simulink model "untitled"  (R2024a)
settings: Solver=FixedStepAuto  StartTime=0.0  StopTime=10  FixedStep=0.001  RelTol=1e-3
values from neighbouring files (symbols this model uses):
  cM = 2.925e-9    (= 2.925e-09)    [untitled1.m]
  CR = 80.584    [untitled1.m]
  cT = 1.4865e-7    (= 1.4865e-07)    [untitled1.m]
  d_x = 0.08257    [untitled1.m]
  d_y = 0.13505    [untitled1.m]
  g = 9.81    [untitled1.m]
  Ix = 0.0095    [untitled1.m]
  Iy = 0.0095    [untitled1.m]
  Iz = 0.019    [untitled1.m]
  K = cM/cT    (= 0.0196770938446)    [untitled1.m]
  Kvxd = 10    [untitled1.m]
  Kvxi = 0.001    [untitled1.m]
  Kvxp = 5    [untitled1.m]
  Kvyd = 10    [untitled1.m]
  Kvyi = 0.001    [untitled1.m]
  Kvyp = 5    [untitled1.m]
  Kvzd = 0.1    [untitled1.m]
  Kvzi = 0.01    [untitled1.m]
  Kvzp = 10    [untitled1.m]
  m = 2    [untitled1.m]
  Tm = 0.03    [untitled1.m]
  wb = 976.2    [untitled1.m]
undefined symbols (not defined in the file or in its folder): Kvpitchd, Kvpitchi, Kvpitchn, Kvpitchp, Kvrolld, Kvrolli, Kvrolln, Kvrollp, Kvyawd, Kvyawi, Kvyawn, Kvyawp, Kzp, magnitude
libraries: slpidlib x6
settings Model: Creator=user  LastModifiedBy=User
settings DataIOCC: ReturnWorkspaceOutputs=off

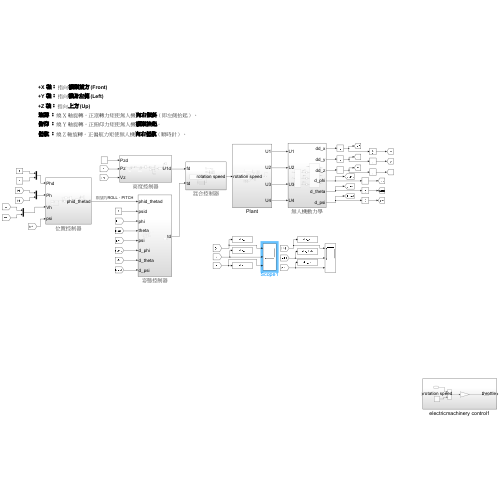
[thumbnail: Simulink's stored preview of the top-level diagram]
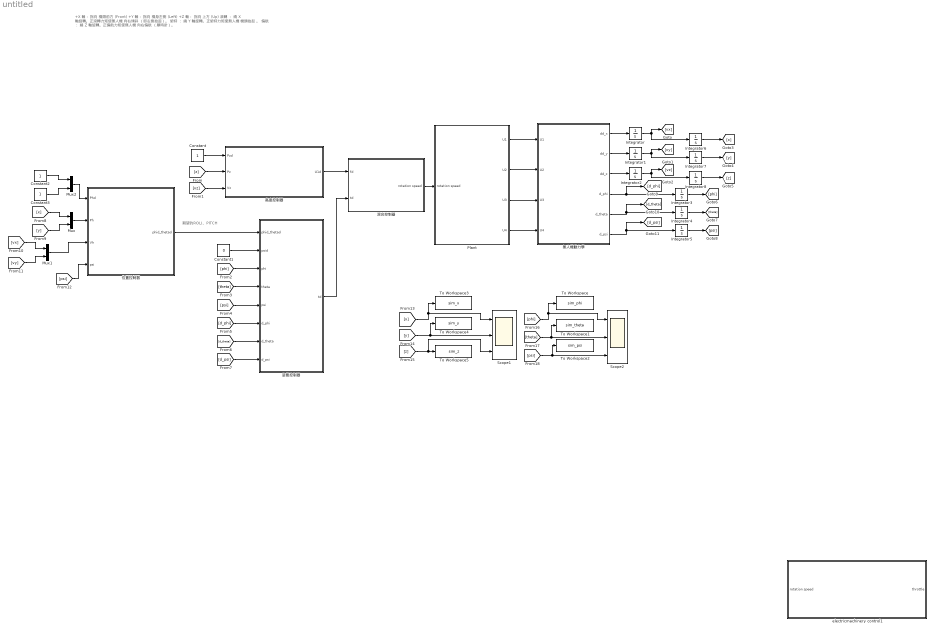
== system untitled ==
  note: +X 軸： 指向 機頭前方 (Front)
      | +Y 軸： 指向 機身左側 (Left)
      | +Z 軸： 指向 上方 (Up)
      | 滾轉 ： 繞 X 軸旋轉。正滾轉力矩使無人機 向右傾斜 （即左側抬起）。
      | 俯仰 ： 繞 Y 軸旋轉。正俯仰力矩使無人機 機頭抬起 。
      | 偏航 ： 繞 Z 軸旋轉。正偏航力矩使無人機 向右偏航 （順時針）。
  note: 期望的ROLL、PITCH
  Constant : Constant
  Constant1 : Constant  Value=0
  Constant2 : Constant
  Constant3 : Constant
  Integrator{,1..8} (9 alike) : Integrator
  Mux : Mux  Inputs=2
  Mux1 : Mux  Inputs=2
  Mux2 : Mux  Inputs=2
  Plant : Subsystem
  Scope1 : Scope  NumInputPorts=3
  Scope2 : Scope  NumInputPorts=3
  To Workspace : ToWorkspace  VariableName=sim_phi  SampleTime=-1
  To Workspace1 : ToWorkspace  VariableName=sim_theta  SampleTime=-1
  To Workspace2 : ToWorkspace  VariableName=sim_psi  SampleTime=-1
  To Workspace3 : ToWorkspace  VariableName=sim_x  SampleTime=-1
  To Workspace4 : ToWorkspace  VariableName=sim_y  SampleTime=-1
  To Workspace5 : ToWorkspace  VariableName=sim_z  SampleTime=-1
  electricmachinery control1 : Subsystem
  位置控制器 : Subsystem
  姿態控制器 : Subsystem
  混合控制器 : Subsystem
  無人機動力學 : Subsystem
  高度控制器 : Subsystem
  wires:
  無人機動力學/1(dd_x) -> Integrator/1
  無人機動力學/2(dd_y) -> Integrator1/1
  無人機動力學/3(dd_z) -> Integrator2/1
  無人機動力學/4(d_phi) -> Integrator3/1, [d_phi]
  無人機動力學/5(d_theta) -> Integrator4/1, [d_theta]
  無人機動力學/6(d_psi) -> Integrator5/1, [d_psi]
  Integrator/1 -> Integrator6/1, [vx]
  Integrator1/1 -> Integrator7/1, [vy]
  Integrator2/1 -> Integrator8/1, [vz]
  Integrator8/1 -> [z]
  Integrator7/1 -> [y]
  Integrator6/1 -> [x]
  Integrator3/1 -> [phi]
  Integrator4/1 -> [theta]
  Integrator5/1 -> [psi]
  高度控制器/1(U1d) -> 混合控制器/1(fd)
  Constant/1 -> 高度控制器/1(Pzd)
  [z] -> 高度控制器/2(Pz)
  [vz] -> 高度控制器/3(Vz)
  位置控制器/1(phid_thetad) -> 姿態控制器/1(phid_thetad)
  Constant1/1 -> 姿態控制器/2(psid)
  [phi] -> 姿態控制器/3(phi)
  [theta] -> 姿態控制器/4(theta)
  [d_psi] -> 姿態控制器/8(d_psi)
  [psi] -> 姿態控制器/5(psi)
  [d_phi] -> 姿態控制器/6(d_phi)
  [d_theta] -> 姿態控制器/7(d_theta)
  姿態控制器/1(td) -> 混合控制器/2(td)
  Mux/1 -> 位置控制器/2(Ph)
  [x] -> Mux/1
  [y] -> Mux/2
  [vx] -> Mux1/1
  [vy] -> Mux1/2
  Mux1/1 -> 位置控制器/3(Vh)
  [psi] -> 位置控制器/4(psi)
  Constant2/1 -> Mux2/1
  Constant3/1 -> Mux2/2
  Mux2/1 -> 位置控制器/1(Phd)
  [y] -> To Workspace4/1, Scope1/2
  [x] -> Scope1/1, To Workspace3/1
  [z] -> To Workspace5/1, Scope1/3
  [phi] -> To Workspace/1, Scope2/1
  [theta] -> To Workspace1/1, Scope2/2
  [psi] -> To Workspace2/1, Scope2/3
  混合控制器/1(rotation speed) -> Plant/1(rotation speed)
  Plant/4(U4) -> 無人機動力學/4(U4)
  Plant/3(U3) -> 無人機動力學/3(U3)
  Plant/2(U2) -> 無人機動力學/2(U2)
  Plant/1(U1) -> 無人機動力學/1(U1)

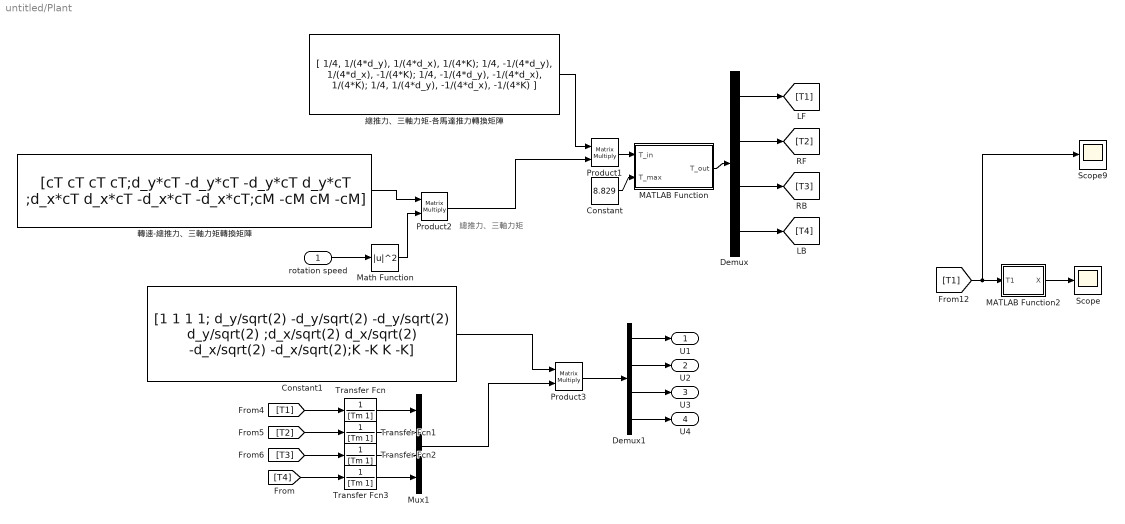
== system untitled/Plant ==
  note: 總推力、三軸力矩
  rotation speed : Inport
  Constant : Constant  Value=8.829
  Constant1 : Constant  Value=[1 1 1 1; d_y/sqrt(2) -d_y/sqrt(2) -d_y/sqrt(2) d_y/sqrt(2) ;d_x/sqrt(2) d_x/sqrt(2) -d_x/sqrt(2) -d_x/sqrt(2);K -K K -K]
  Demux : Demux
  Demux1 : Demux
  MATLAB Function : MATLAB Function  TreatAsAtomicUnit=on
  MATLAB Function2 : MATLAB Function  TreatAsAtomicUnit=on
  Math Function : Math  Operator=magnitude^2
  Mux1 : Mux
  Product1 : Product  Multiplication=Matrix(*)
  Product2 : Product  Multiplication=Matrix(*)
  Product3 : Product  Multiplication=Matrix(*)
  Scope : Scope
  Scope9 : Scope
  Transfer Fcn{,1..3} (4 alike) : TransferFcn  Denominator=[Tm 1]
  總推力、三軸力矩-各馬達推力轉換矩陣 : Constant  Value=|
      | [ 1/4,    1/(4*d_y),    1/(4*d_x),    1/(4*K);
      |   1/4,   -1/(4*d_y),    1/(4*d_x),   -1/(4*K);
      |   1/4,   -1/(4*d_y),   -1/(4*d_x),    1/(4*K);
      |   1/4,    1/(4*d_y),   -1/(4*d_x),   -1/(4*K) ]
  轉速-總推力、三軸力矩轉換矩陣 : Constant  Value=[cT cT cT cT;d_y*cT -d_y*cT -d_y*cT d_y*cT ;d_x*cT d_x*cT -d_x*cT -d_x*cT;cM -cM cM -cM]
  U1 : Outport
  U2 : Outport  Port=2
  U3 : Outport  Port=3
  U4 : Outport  Port=4
  wires:
  Constant1/1 -> Product3/1
  [T1] -> Scope9/1, MATLAB Function2/1(T1)
  MATLAB Function2/1(X) -> Scope/1
  Product3/1 -> Demux1/1
  Demux1/3 -> U3/1
  Demux1/4 -> U4/1
  Demux1/1 -> U1/1
  Demux1/2 -> U2/1
  Demux/1 -> [T1]
  Demux/2 -> [T2]
  Demux/3 -> [T3]
  Demux/4 -> [T4]
  總推力、三軸力矩-各馬達推力轉換矩陣/1 -> Product1/1
  轉速-總推力、三軸力矩轉換矩陣/1 -> Product2/1
  Transfer Fcn/1 -> Mux1/1
  Transfer Fcn1/1 -> Mux1/2
  Transfer Fcn2/1 -> Mux1/3
  Transfer Fcn3/1 -> Mux1/4
  Product2/1 -> Product1/2
  rotation speed/1 -> Math Function/1
  [T1] -> Transfer Fcn/1
  [T2] -> Transfer Fcn1/1
  [T3] -> Transfer Fcn2/1
  [T4] -> Transfer Fcn3/1
  Math Function/1 -> Product2/2
  Mux1/1 -> Product3/2
  MATLAB Function/1(T_out) -> Demux/1
  Product1/1 -> MATLAB Function/1(T_in)
  Constant/1 -> MATLAB Function/2(T_max)

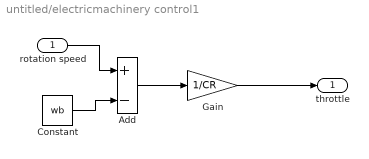
== system untitled/electricmachinery control1 ==
  rotation speed : Inport
  Add : Sum  Inputs=+-
  Constant : Constant  Value=wb
  Gain : Gain  Gain=1/CR
  throttle : Outport
  wires:
  Add/1 -> Gain/1
  rotation speed/1 -> Add/1
  Constant/1 -> Add/2
  Gain/1 -> throttle/1

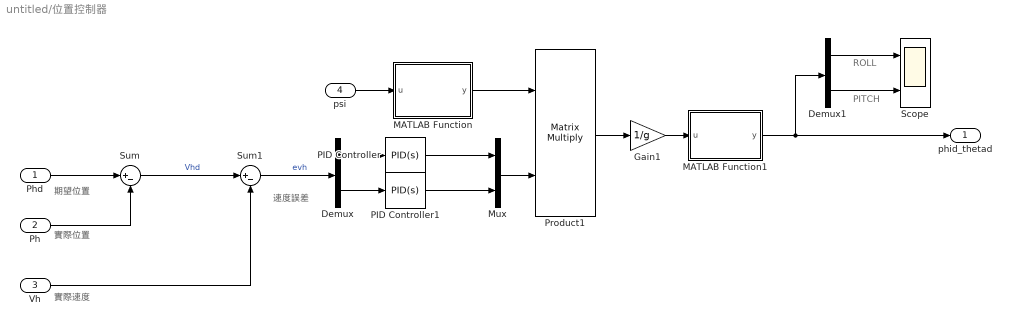
== system untitled/位置控制器 ==
  note: ROLL
  note: 期望位置
  note: 實際位置
  note: 實際速度
  note: 速度誤差
  note: PITCH
  Phd : Inport
  Ph : Inport  Port=2
  Vh : Inport  Port=3
  psi : Inport  Port=4
  Demux : Demux  Outputs=2
  Demux1 : Demux  Outputs=2
  Gain1 : Gain  Gain=1/g
  MATLAB Function : MATLAB Function  TreatAsAtomicUnit=on
  MATLAB Function1 : MATLAB Function  TreatAsAtomicUnit=on
  Mux : Mux  Inputs=2
  PID Controller : slpidlib/PID Controller  Controller=PID  Form=Parallel  TimeDomain=Continuous-time  UseExternalTs=off  SampleTime=-1  IntegratorMethod=Forward Euler  FilterMethod=Forward Euler  ControllerParametersSource=internal  P=Kvxp  I=Kvxi  UseKiTs=off  D=Kvxd  UseExternalDerivativeSource=off  N=100  UseFilter=on  TunerSelectOption=Transfer Function Based (PID Tuner App)  InitialConditionSource=internal  InitialConditionForIntegrator=0  InitialConditionForFilter=0  DifferentiatorICPrevScaledInput=0  ExternalReset=none  TrackingMode=off  Kt=1  LimitOutput=off  SatLimitsSource=internal  UpperSaturationLimit=inf  LowerSaturationLimit=-inf  LinearizeAsGain=on  AntiWindupMode=none  Kb=1  LimitIntegrator=off  UpperIntegratorSaturationLimit=inf  LowerIntegratorSaturationLimit=-inf  POutMin=[]  POutMax=[]  IOutMin=[]  IOutMax=[]  DOutMin=[]  DOutMax=[]  NOutMin=[]  NOutMax=[]  SumOutMin=[]  SumOutMax=[]  SaturationOutMin=[]  SaturationOutMax=[]  PParamMin=[]  PParamMax=[]  IParamMin=[]  IParamMax=[]  DParamMin=[]  DParamMax=[]  NParamMin=[]  NParamMax=[]  KbParamMin=[]  KbParamMax=[]  KtParamMin=[]  KtParamMax=[]  KbOutMin=[]  KbOutMax=[]  KtOutMin=[]  KtOutMax=[]  IntegratorOutMin=[]  IntegratorOutMax=[]  FilterOutMin=[]  FilterOutMax=[]  SumI1OutMin=[]  SumI1OutMax=[]  SumI2OutMin=[]  SumI2OutMax=[]  SumI3OutMin=[]  SumI3OutMax=[]  SumI4OutMin=[]  SumI4OutMax=[]  SumDOutMin=[]  SumDOutMax=[]  DifferentiatorOutMin=[]  DifferentiatorOutMax=[]  FilterDiffOutCoefMin=[]  FilterDiffOutCoefMax=[]  ReciprocalOutMin=[]  ReciprocalOutMax=[]  SumDenOutMin=[]  SumDenOutMax=[]  SumNumOutMin=[]  SumNumOutMax=[]  DivideOutMin=[]  DivideOutMax=[]  UdiffTsProdOutMin=[]  UdiffTsProdOutMax=[]  NTsProdOutMin=[]  NTsProdOutMax=[]  UintegralTsProdOutMin=[]  UintegralTsProdOutMax=[]  UngainTsProdOutMin=[]  UngainTsProdOutMax=[]  ClampingZeroOutDataTypeStr=Inherit: Inherit via back propagation  ClampingZeroOutMin=[]  ClampingZeroOutMax=[]  FilterDenConstantOutDataTypeStr=Inherit: Inherit via back propagation  FilterDenConstantOutMin=[]  FilterDenConstantOutMax=[]  PCopyOutDataTypeStr=Inherit: Inherit via back propagation  PCopyOutMin=[]  PCopyOutMax=[]  NCopyOutDataTypeStr=Inherit: Inherit via back propagation  NCopyOutMin=[]  NCopyOutMax=[]  IntegratorContinuousStateAttributes=''  IntegratorStateMustResolveToSignalObject=off  IntegratorRTWStateStorageClass=Auto  FilterContinuousStateAttributes=''  FilterStateMustResolveToSignalObject=off  FilterRTWStateStorageClass=Auto  ParallelPVariant=InternalParameters  IdealPVariant=Disabled  IVariant=InternalParameters  DVariant=InternalParameters  IntegratorVariant=Continuous  SatVariant=Disabled  AWVariant=Passthrough  PCopyVariant=Disabled  TRVariant=Disabled  FdbkBlocksVariant=Forward  IdealPFdbkVariant=Disabled  SatFdbkVariant=Disabled  DerivativeFilterVariant=ContFilter  NVariant=InternalParameters  NCopyVariant=Disabled  FilterICVariant=InternalICsFilter  IntegratorICVariant=InternalICs  ExternalResetVariant=Disabled  TRSumVariant=Passthrough  SumFdbkVariant=Disabled  SumVariant=Sum_PID  TsampFilterVariant=InternalTs  TsampNgainVariant=Passthrough  TsampIntegralVariant=Disabled_SignalSpec  ExternalSaturationOutDataTypeStr=Inherit: Same as second input  DerivativeSourceVariant=ErrorSignal
  PID Controller1 : slpidlib/PID Controller  Controller=PID  Form=Parallel  TimeDomain=Continuous-time  UseExternalTs=off  SampleTime=-1  IntegratorMethod=Forward Euler  FilterMethod=Forward Euler  ControllerParametersSource=internal  P=Kvyp  I=Kvyi  UseKiTs=off  D=Kvyd  UseExternalDerivativeSource=off  N=100  UseFilter=on  TunerSelectOption=Transfer Function Based (PID Tuner App)  InitialConditionSource=internal  InitialConditionForIntegrator=0  InitialConditionForFilter=0  DifferentiatorICPrevScaledInput=0  ExternalReset=none  TrackingMode=off  Kt=1  LimitOutput=off  SatLimitsSource=internal  UpperSaturationLimit=inf  LowerSaturationLimit=-inf  LinearizeAsGain=on  AntiWindupMode=none  Kb=1  LimitIntegrator=off  UpperIntegratorSaturationLimit=inf  LowerIntegratorSaturationLimit=-inf  POutMin=[]  POutMax=[]  IOutMin=[]  IOutMax=[]  DOutMin=[]  DOutMax=[]  NOutMin=[]  NOutMax=[]  SumOutMin=[]  SumOutMax=[]  SaturationOutMin=[]  SaturationOutMax=[]  PParamMin=[]  PParamMax=[]  IParamMin=[]  IParamMax=[]  DParamMin=[]  DParamMax=[]  NParamMin=[]  NParamMax=[]  KbParamMin=[]  KbParamMax=[]  KtParamMin=[]  KtParamMax=[]  KbOutMin=[]  KbOutMax=[]  KtOutMin=[]  KtOutMax=[]  IntegratorOutMin=[]  IntegratorOutMax=[]  FilterOutMin=[]  FilterOutMax=[]  SumI1OutMin=[]  SumI1OutMax=[]  SumI2OutMin=[]  SumI2OutMax=[]  SumI3OutMin=[]  SumI3OutMax=[]  SumI4OutMin=[]  SumI4OutMax=[]  SumDOutMin=[]  SumDOutMax=[]  DifferentiatorOutMin=[]  DifferentiatorOutMax=[]  FilterDiffOutCoefMin=[]  FilterDiffOutCoefMax=[]  ReciprocalOutMin=[]  ReciprocalOutMax=[]  SumDenOutMin=[]  SumDenOutMax=[]  SumNumOutMin=[]  SumNumOutMax=[]  DivideOutMin=[]  DivideOutMax=[]  UdiffTsProdOutMin=[]  UdiffTsProdOutMax=[]  NTsProdOutMin=[]  NTsProdOutMax=[]  UintegralTsProdOutMin=[]  UintegralTsProdOutMax=[]  UngainTsProdOutMin=[]  UngainTsProdOutMax=[]  ClampingZeroOutDataTypeStr=Inherit: Inherit via back propagation  ClampingZeroOutMin=[]  ClampingZeroOutMax=[]  FilterDenConstantOutDataTypeStr=Inherit: Inherit via back propagation  FilterDenConstantOutMin=[]  FilterDenConstantOutMax=[]  PCopyOutDataTypeStr=Inherit: Inherit via back propagation  PCopyOutMin=[]  PCopyOutMax=[]  NCopyOutDataTypeStr=Inherit: Inherit via back propagation  NCopyOutMin=[]  NCopyOutMax=[]  IntegratorContinuousStateAttributes=''  IntegratorStateMustResolveToSignalObject=off  IntegratorRTWStateStorageClass=Auto  FilterContinuousStateAttributes=''  FilterStateMustResolveToSignalObject=off  FilterRTWStateStorageClass=Auto  ParallelPVariant=InternalParameters  IdealPVariant=Disabled  IVariant=InternalParameters  DVariant=InternalParameters  IntegratorVariant=Continuous  SatVariant=Disabled  AWVariant=Passthrough  PCopyVariant=Disabled  TRVariant=Disabled  FdbkBlocksVariant=Forward  IdealPFdbkVariant=Disabled  SatFdbkVariant=Disabled  DerivativeFilterVariant=ContFilter  NVariant=InternalParameters  NCopyVariant=Disabled  FilterICVariant=InternalICsFilter  IntegratorICVariant=InternalICs  ExternalResetVariant=Disabled  TRSumVariant=Passthrough  SumFdbkVariant=Disabled  SumVariant=Sum_PID  TsampFilterVariant=InternalTs  TsampNgainVariant=Passthrough  TsampIntegralVariant=Disabled_SignalSpec  ExternalSaturationOutDataTypeStr=Inherit: Same as second input  DerivativeSourceVariant=ErrorSignal
  Product1 : Product  Multiplication=Matrix(*)
  Scope : Scope  NumInputPorts=2
  Sum : Sum  Inputs=|+-
  Sum1 : Sum  Inputs=|+-
  phid_thetad : Outport
  wires:
  Gain1/1 -> MATLAB Function1/1(u)
  Phd/1 -> Sum/1
  Demux/1 -> PID Controller/1
  Ph/1 -> Sum/2
  psi/1 -> MATLAB Function/1(u)
  Product1/1 -> Gain1/1
  PID Controller/1 -> Mux/1
  Demux/2 -> PID Controller1/1
  Sum1/1 -> Demux/1  "evh"
  Mux/1 -> Product1/2
  Vh/1 -> Sum1/2
  Sum/1 -> Sum1/1  "Vhd"
  MATLAB Function1/1(y) -> Demux1/1, phid_thetad/1
  MATLAB Function/1(y) -> Product1/1
  PID Controller1/1 -> Mux/2
  Demux1/1 -> Scope/1
  Demux1/2 -> Scope/2

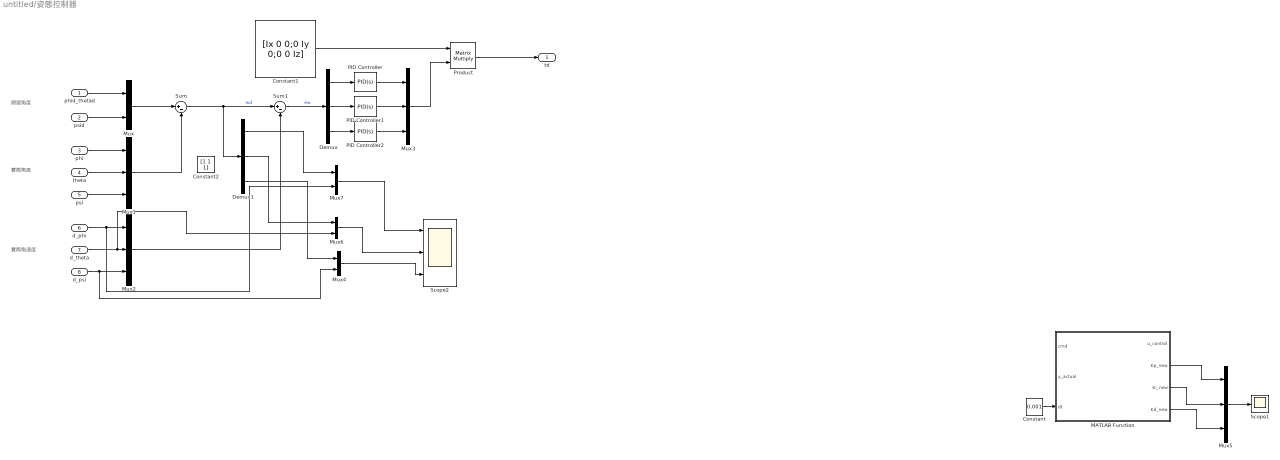
== system untitled/姿態控制器 ==
  note: 實際角速度
  note: 實際角度
  note: 期望角度
  phid_thetad : Inport
  psid : Inport  Port=2
  phi : Inport  Port=3
  theta : Inport  Port=4
  psi : Inport  Port=5
  d_phi : Inport  Port=6
  d_theta : Inport  Port=7
  d_psi : Inport  Port=8
  Constant : Constant  Value=0.001
  Constant1 : Constant  Value=[Ix 0 0;0 Iy 0;0 0 Iz]
  Constant2 : Constant  Value=[1 1 1]
  Demux : Demux  Outputs=3
  Demux1 : Demux  Outputs=3
  MATLAB Function : MATLAB Function  TreatAsAtomicUnit=on
  Mux{,4,6..7} (4 alike) : Mux  Inputs=2
  Mux{1..3,5} (4 alike) : Mux  Inputs=3
  PID Controller : slpidlib/PID Controller  Controller=PID  Form=Parallel  TimeDomain=Continuous-time  UseExternalTs=off  SampleTime=-1  IntegratorMethod=Forward Euler  FilterMethod=Forward Euler  ControllerParametersSource=internal  P=Kvrollp  I=Kvrolli  UseKiTs=off  D=Kvrolld  UseExternalDerivativeSource=off  N=Kvrolln  UseFilter=on  TunerSelectOption=Transfer Function Based (PID Tuner App)  InitialConditionSource=internal  InitialConditionForIntegrator=0  InitialConditionForFilter=0  DifferentiatorICPrevScaledInput=0  ExternalReset=none  TrackingMode=off  Kt=1  LimitOutput=off  SatLimitsSource=internal  UpperSaturationLimit=inf  LowerSaturationLimit=-inf  LinearizeAsGain=on  AntiWindupMode=none  Kb=1  LimitIntegrator=off  UpperIntegratorSaturationLimit=inf  LowerIntegratorSaturationLimit=-inf  POutMin=[]  POutMax=[]  IOutMin=[]  IOutMax=[]  DOutMin=[]  DOutMax=[]  NOutMin=[]  NOutMax=[]  SumOutMin=[]  SumOutMax=[]  SaturationOutMin=[]  SaturationOutMax=[]  PParamMin=[]  PParamMax=[]  IParamMin=[]  IParamMax=[]  DParamMin=[]  DParamMax=[]  NParamMin=[]  NParamMax=[]  KbParamMin=[]  KbParamMax=[]  KtParamMin=[]  KtParamMax=[]  KbOutMin=[]  KbOutMax=[]  KtOutMin=[]  KtOutMax=[]  IntegratorOutMin=[]  IntegratorOutMax=[]  FilterOutMin=[]  FilterOutMax=[]  SumI1OutMin=[]  SumI1OutMax=[]  SumI2OutMin=[]  SumI2OutMax=[]  SumI3OutMin=[]  SumI3OutMax=[]  SumI4OutMin=[]  SumI4OutMax=[]  SumDOutMin=[]  SumDOutMax=[]  DifferentiatorOutMin=[]  DifferentiatorOutMax=[]  FilterDiffOutCoefMin=[]  FilterDiffOutCoefMax=[]  ReciprocalOutMin=[]  ReciprocalOutMax=[]  SumDenOutMin=[]  SumDenOutMax=[]  SumNumOutMin=[]  SumNumOutMax=[]  DivideOutMin=[]  DivideOutMax=[]  UdiffTsProdOutMin=[]  UdiffTsProdOutMax=[]  NTsProdOutMin=[]  NTsProdOutMax=[]  UintegralTsProdOutMin=[]  UintegralTsProdOutMax=[]  UngainTsProdOutMin=[]  UngainTsProdOutMax=[]  ClampingZeroOutDataTypeStr=Inherit: Inherit via back propagation  ClampingZeroOutMin=[]  ClampingZeroOutMax=[]  FilterDenConstantOutDataTypeStr=Inherit: Inherit via back propagation  FilterDenConstantOutMin=[]  FilterDenConstantOutMax=[]  PCopyOutDataTypeStr=Inherit: Inherit via back propagation  PCopyOutMin=[]  PCopyOutMax=[]  NCopyOutDataTypeStr=Inherit: Inherit via back propagation  NCopyOutMin=[]  NCopyOutMax=[]  IntegratorContinuousStateAttributes=''  IntegratorStateMustResolveToSignalObject=off  IntegratorRTWStateStorageClass=Auto  FilterContinuousStateAttributes=''  FilterStateMustResolveToSignalObject=off  FilterRTWStateStorageClass=Auto  ParallelPVariant=InternalParameters  IdealPVariant=Disabled  IVariant=InternalParameters  DVariant=InternalParameters  IntegratorVariant=Continuous  SatVariant=Disabled  AWVariant=Passthrough  PCopyVariant=Disabled  TRVariant=Disabled  FdbkBlocksVariant=Forward  IdealPFdbkVariant=Disabled  SatFdbkVariant=Disabled  DerivativeFilterVariant=ContFilter  NVariant=InternalParameters  NCopyVariant=Disabled  FilterICVariant=InternalICsFilter  IntegratorICVariant=InternalICs  ExternalResetVariant=Disabled  TRSumVariant=Passthrough  SumFdbkVariant=Disabled  SumVariant=Sum_PID  TsampFilterVariant=InternalTs  TsampNgainVariant=Passthrough  TsampIntegralVariant=Disabled_SignalSpec  ExternalSaturationOutDataTypeStr=Inherit: Same as second input  DerivativeSourceVariant=ErrorSignal
  PID Controller1 : slpidlib/PID Controller  Controller=PID  Form=Parallel  TimeDomain=Continuous-time  UseExternalTs=off  SampleTime=-1  IntegratorMethod=Forward Euler  FilterMethod=Forward Euler  ControllerParametersSource=internal  P=Kvpitchp  I=Kvpitchi  UseKiTs=off  D=Kvpitchd  UseExternalDerivativeSource=off  N=Kvpitchn  UseFilter=on  TunerSelectOption=Transfer Function Based (PID Tuner App)  InitialConditionSource=internal  InitialConditionForIntegrator=0  InitialConditionForFilter=0  DifferentiatorICPrevScaledInput=0  ExternalReset=none  TrackingMode=off  Kt=1  LimitOutput=off  SatLimitsSource=internal  UpperSaturationLimit=inf  LowerSaturationLimit=-inf  LinearizeAsGain=on  AntiWindupMode=none  Kb=1  LimitIntegrator=off  UpperIntegratorSaturationLimit=inf  LowerIntegratorSaturationLimit=-inf  POutMin=[]  POutMax=[]  IOutMin=[]  IOutMax=[]  DOutMin=[]  DOutMax=[]  NOutMin=[]  NOutMax=[]  SumOutMin=[]  SumOutMax=[]  SaturationOutMin=[]  SaturationOutMax=[]  PParamMin=[]  PParamMax=[]  IParamMin=[]  IParamMax=[]  DParamMin=[]  DParamMax=[]  NParamMin=[]  NParamMax=[]  KbParamMin=[]  KbParamMax=[]  KtParamMin=[]  KtParamMax=[]  KbOutMin=[]  KbOutMax=[]  KtOutMin=[]  KtOutMax=[]  IntegratorOutMin=[]  IntegratorOutMax=[]  FilterOutMin=[]  FilterOutMax=[]  SumI1OutMin=[]  SumI1OutMax=[]  SumI2OutMin=[]  SumI2OutMax=[]  SumI3OutMin=[]  SumI3OutMax=[]  SumI4OutMin=[]  SumI4OutMax=[]  SumDOutMin=[]  SumDOutMax=[]  DifferentiatorOutMin=[]  DifferentiatorOutMax=[]  FilterDiffOutCoefMin=[]  FilterDiffOutCoefMax=[]  ReciprocalOutMin=[]  ReciprocalOutMax=[]  SumDenOutMin=[]  SumDenOutMax=[]  SumNumOutMin=[]  SumNumOutMax=[]  DivideOutMin=[]  DivideOutMax=[]  UdiffTsProdOutMin=[]  UdiffTsProdOutMax=[]  NTsProdOutMin=[]  NTsProdOutMax=[]  UintegralTsProdOutMin=[]  UintegralTsProdOutMax=[]  UngainTsProdOutMin=[]  UngainTsProdOutMax=[]  ClampingZeroOutDataTypeStr=Inherit: Inherit via back propagation  ClampingZeroOutMin=[]  ClampingZeroOutMax=[]  FilterDenConstantOutDataTypeStr=Inherit: Inherit via back propagation  FilterDenConstantOutMin=[]  FilterDenConstantOutMax=[]  PCopyOutDataTypeStr=Inherit: Inherit via back propagation  PCopyOutMin=[]  PCopyOutMax=[]  NCopyOutDataTypeStr=Inherit: Inherit via back propagation  NCopyOutMin=[]  NCopyOutMax=[]  IntegratorContinuousStateAttributes=''  IntegratorStateMustResolveToSignalObject=off  IntegratorRTWStateStorageClass=Auto  FilterContinuousStateAttributes=''  FilterStateMustResolveToSignalObject=off  FilterRTWStateStorageClass=Auto  ParallelPVariant=InternalParameters  IdealPVariant=Disabled  IVariant=InternalParameters  DVariant=InternalParameters  IntegratorVariant=Continuous  SatVariant=Disabled  AWVariant=Passthrough  PCopyVariant=Disabled  TRVariant=Disabled  FdbkBlocksVariant=Forward  IdealPFdbkVariant=Disabled  SatFdbkVariant=Disabled  DerivativeFilterVariant=ContFilter  NVariant=InternalParameters  NCopyVariant=Disabled  FilterICVariant=InternalICsFilter  IntegratorICVariant=InternalICs  ExternalResetVariant=Disabled  TRSumVariant=Passthrough  SumFdbkVariant=Disabled  SumVariant=Sum_PID  TsampFilterVariant=InternalTs  TsampNgainVariant=Passthrough  TsampIntegralVariant=Disabled_SignalSpec  ExternalSaturationOutDataTypeStr=Inherit: Same as second input  DerivativeSourceVariant=ErrorSignal
  PID Controller2 : slpidlib/PID Controller  Controller=PID  Form=Parallel  TimeDomain=Continuous-time  UseExternalTs=off  SampleTime=-1  IntegratorMethod=Forward Euler  FilterMethod=Forward Euler  ControllerParametersSource=internal  P=Kvyawp  I=Kvyawi  UseKiTs=off  D=Kvyawd  UseExternalDerivativeSource=off  N=Kvyawn  UseFilter=on  TunerSelectOption=Transfer Function Based (PID Tuner App)  InitialConditionSource=internal  InitialConditionForIntegrator=0  InitialConditionForFilter=0  DifferentiatorICPrevScaledInput=0  ExternalReset=none  TrackingMode=off  Kt=1  LimitOutput=on  SatLimitsSource=internal  UpperSaturationLimit=3  LowerSaturationLimit=-3  LinearizeAsGain=on  AntiWindupMode=none  Kb=1  LimitIntegrator=off  UpperIntegratorSaturationLimit=inf  LowerIntegratorSaturationLimit=-inf  POutMin=[]  POutMax=[]  IOutMin=[]  IOutMax=[]  DOutMin=[]  DOutMax=[]  NOutMin=[]  NOutMax=[]  SumOutMin=[]  SumOutMax=[]  SaturationOutMin=[]  SaturationOutMax=[]  PParamMin=[]  PParamMax=[]  IParamMin=[]  IParamMax=[]  DParamMin=[]  DParamMax=[]  NParamMin=[]  NParamMax=[]  KbParamMin=[]  KbParamMax=[]  KtParamMin=[]  KtParamMax=[]  KbOutMin=[]  KbOutMax=[]  KtOutMin=[]  KtOutMax=[]  IntegratorOutMin=[]  IntegratorOutMax=[]  FilterOutMin=[]  FilterOutMax=[]  SumI1OutMin=[]  SumI1OutMax=[]  SumI2OutMin=[]  SumI2OutMax=[]  SumI3OutMin=[]  SumI3OutMax=[]  SumI4OutMin=[]  SumI4OutMax=[]  SumDOutMin=[]  SumDOutMax=[]  DifferentiatorOutMin=[]  DifferentiatorOutMax=[]  FilterDiffOutCoefMin=[]  FilterDiffOutCoefMax=[]  ReciprocalOutMin=[]  ReciprocalOutMax=[]  SumDenOutMin=[]  SumDenOutMax=[]  SumNumOutMin=[]  SumNumOutMax=[]  DivideOutMin=[]  DivideOutMax=[]  UdiffTsProdOutMin=[]  UdiffTsProdOutMax=[]  NTsProdOutMin=[]  NTsProdOutMax=[]  UintegralTsProdOutMin=[]  UintegralTsProdOutMax=[]  UngainTsProdOutMin=[]  UngainTsProdOutMax=[]  ClampingZeroOutDataTypeStr=Inherit: Inherit via back propagation  ClampingZeroOutMin=[]  ClampingZeroOutMax=[]  FilterDenConstantOutDataTypeStr=Inherit: Inherit via back propagation  FilterDenConstantOutMin=[]  FilterDenConstantOutMax=[]  PCopyOutDataTypeStr=Inherit: Inherit via back propagation  PCopyOutMin=[]  PCopyOutMax=[]  NCopyOutDataTypeStr=Inherit: Inherit via back propagation  NCopyOutMin=[]  NCopyOutMax=[]  IntegratorContinuousStateAttributes=''  IntegratorStateMustResolveToSignalObject=off  IntegratorRTWStateStorageClass=Auto  FilterContinuousStateAttributes=''  FilterStateMustResolveToSignalObject=off  FilterRTWStateStorageClass=Auto  ParallelPVariant=InternalParameters  IdealPVariant=Disabled  IVariant=InternalParameters  DVariant=InternalParameters  IntegratorVariant=Continuous  SatVariant=Enabled  AWVariant=Passthrough  PCopyVariant=Disabled  TRVariant=Disabled  FdbkBlocksVariant=Forward  IdealPFdbkVariant=Disabled  SatFdbkVariant=Disabled  DerivativeFilterVariant=ContFilter  NVariant=InternalParameters  NCopyVariant=Disabled  FilterICVariant=InternalICsFilter  IntegratorICVariant=InternalICs  ExternalResetVariant=Disabled  TRSumVariant=Passthrough  SumFdbkVariant=Disabled  SumVariant=Sum_PID  TsampFilterVariant=InternalTs  TsampNgainVariant=Passthrough  TsampIntegralVariant=Disabled_SignalSpec  ExternalSaturationOutDataTypeStr=Inherit: Same as second input  DerivativeSourceVariant=ErrorSignal
  Product : Product  Multiplication=Matrix(*)
  Scope1 : Scope
  Scope2 : Scope  NumInputPorts=3
  Sum : Sum  Inputs=|+-
  Sum1 : Sum  Inputs=|+-
  td : Outport
  wires:
  phid_thetad/1 -> Mux/1
  Demux/2 -> PID Controller1/1
  Demux/3 -> PID Controller2/1
  psi/1 -> Mux1/3
  phi/1 -> Mux1/1
  psid/1 -> Mux/2
  Sum1/1 -> Demux/1  "ew"
  Mux/1 -> Sum/1
  Mux3/1 -> Product/2
  theta/1 -> Mux1/2
  Product/1 -> td/1
  Mux1/1 -> Sum/2
  PID Controller1/1 -> Mux3/2
  d_psi/1 -> Mux4/2, Mux2/3
  PID Controller2/1 -> Mux3/3
  Constant1/1 -> Product/1
  d_theta/1 -> Mux6/2, Mux2/2
  Mux2/1 -> Sum1/2
  Sum/1 -> Demux1/1, Sum1/1  "wd"
  Constant/1 -> MATLAB Function/3(dt)
  Mux5/1 -> Scope1/1
  MATLAB Function/2(Kp_new) -> Mux5/1
  MATLAB Function/3(Ki_new) -> Mux5/2
  MATLAB Function/4(Kd_new) -> Mux5/3
  Demux/1 -> PID Controller/1
  PID Controller/1 -> Mux3/1
  Mux4/1 -> Scope2/3
  Demux1/3 -> Mux4/1
  Mux6/1 -> Scope2/2
  Mux7/1 -> Scope2/1
  Demux1/1 -> Mux7/1
  Demux1/2 -> Mux6/1
  d_phi/1 -> Mux7/2, Mux2/1

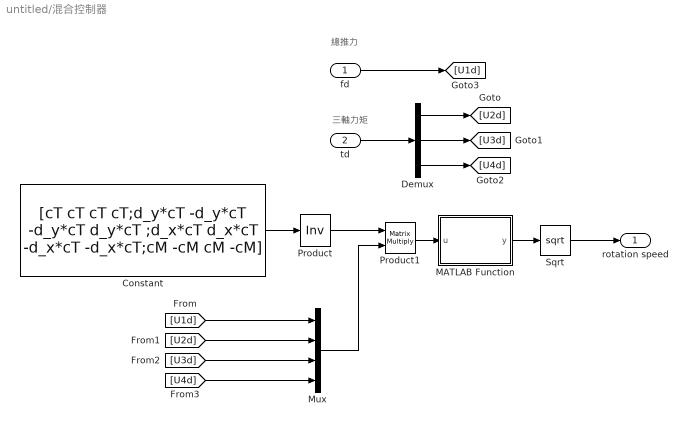
== system untitled/混合控制器 ==
  note: 三軸力矩
  note: 總推力
  fd : Inport
  td : Inport  Port=2
  Constant : Constant  Value=[cT cT cT cT;d_y*cT -d_y*cT -d_y*cT d_y*cT ;d_x*cT d_x*cT -d_x*cT -d_x*cT;cM -cM cM -cM]
  Demux : Demux  Outputs=3
  MATLAB Function : MATLAB Function  TreatAsAtomicUnit=on
  Mux : Mux
  Product : Product  Inputs=/  Multiplication=Matrix(*)
  Product1 : Product  Multiplication=Matrix(*)
  Sqrt : Sqrt
  rotation speed : Outport
  wires:
  [U4d] -> Mux/4
  td/1 -> Demux/1
  Constant/1 -> Product/1
  Mux/1 -> Product1/2
  Demux/1 -> [U2d]
  [U3d] -> Mux/3
  [U2d] -> Mux/2
  Product/1 -> Product1/1
  fd/1 -> [U1d]
  Demux/3 -> [U4d]
  Demux/2 -> [U3d]
  [U1d] -> Mux/1
  Sqrt/1 -> rotation speed/1
  Product1/1 -> MATLAB Function/1(u)
  MATLAB Function/1(y) -> Sqrt/1

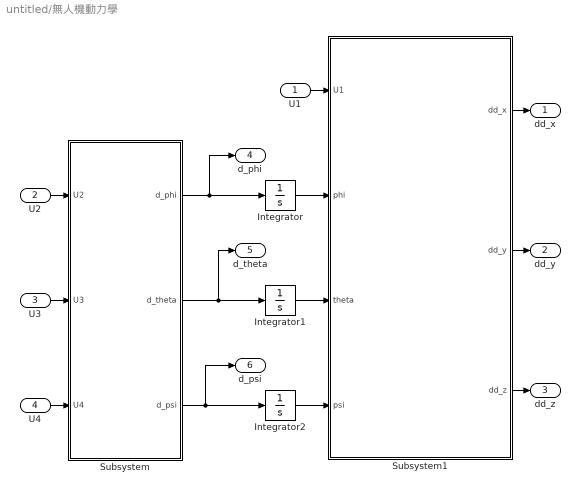
== system untitled/無人機動力學 ==
  U1 : Inport
  U2 : Inport  Port=2
  U3 : Inport  Port=3
  U4 : Inport  Port=4
  Integrator : Integrator
  Integrator1 : Integrator
  Integrator2 : Integrator
  Subsystem : Subsystem
  Subsystem1 : Subsystem
  dd_x : Outport
  dd_y : Outport  Port=2
  dd_z : Outport  Port=3
  d_phi : Outport  Port=4
  d_theta : Outport  Port=5
  d_psi : Outport  Port=6
  wires:
  Integrator1/1 -> Subsystem1/3(theta)
  Subsystem/3(d_psi) -> d_psi/1, Integrator2/1
  Subsystem/2(d_theta) -> d_theta/1, Integrator1/1
  Subsystem1/1(dd_x) -> dd_x/1
  Integrator/1 -> Subsystem1/2(phi)
  U3/1 -> Subsystem/2(U3)
  Subsystem/1(d_phi) -> d_phi/1, Integrator/1
  Integrator2/1 -> Subsystem1/4(psi)
  U4/1 -> Subsystem/3(U4)
  Subsystem1/2(dd_y) -> dd_y/1
  Subsystem1/3(dd_z) -> dd_z/1
  U1/1 -> Subsystem1/1(U1)
  U2/1 -> Subsystem/1(U2)

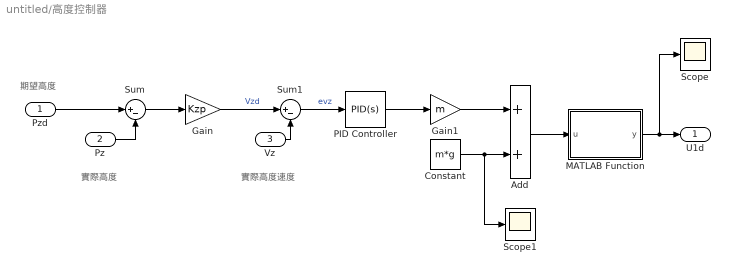
== system untitled/高度控制器 ==
  note: 期望高度
  note: 實際高度
  note: 實際高度速度
  Pzd : Inport
  Pz : Inport  Port=2
  Vz : Inport  Port=3
  Add : Sum
  Constant : Constant  Value=m*g
  Gain : Gain  Gain=Kzp
  Gain1 : Gain  Gain=m
  MATLAB Function : MATLAB Function  TreatAsAtomicUnit=on
  PID Controller : slpidlib/PID Controller  Controller=PID  Form=Parallel  TimeDomain=Continuous-time  UseExternalTs=off  SampleTime=-1  IntegratorMethod=Forward Euler  FilterMethod=Forward Euler  ControllerParametersSource=internal  P=Kvzp  I=Kvzi  UseKiTs=off  D=Kvzd  UseExternalDerivativeSource=off  N=100  UseFilter=on  TunerSelectOption=Transfer Function Based (PID Tuner App)  InitialConditionSource=internal  InitialConditionForIntegrator=0  InitialConditionForFilter=0  DifferentiatorICPrevScaledInput=0  ExternalReset=none  TrackingMode=off  Kt=1  LimitOutput=off  SatLimitsSource=internal  UpperSaturationLimit=inf  LowerSaturationLimit=-inf  LinearizeAsGain=on  AntiWindupMode=none  Kb=1  LimitIntegrator=off  UpperIntegratorSaturationLimit=inf  LowerIntegratorSaturationLimit=-inf  POutMin=[]  POutMax=[]  IOutMin=[]  IOutMax=[]  DOutMin=[]  DOutMax=[]  NOutMin=[]  NOutMax=[]  SumOutMin=[]  SumOutMax=[]  SaturationOutMin=[]  SaturationOutMax=[]  PParamMin=[]  PParamMax=[]  IParamMin=[]  IParamMax=[]  DParamMin=[]  DParamMax=[]  NParamMin=[]  NParamMax=[]  KbParamMin=[]  KbParamMax=[]  KtParamMin=[]  KtParamMax=[]  KbOutMin=[]  KbOutMax=[]  KtOutMin=[]  KtOutMax=[]  IntegratorOutMin=[]  IntegratorOutMax=[]  FilterOutMin=[]  FilterOutMax=[]  SumI1OutMin=[]  SumI1OutMax=[]  SumI2OutMin=[]  SumI2OutMax=[]  SumI3OutMin=[]  SumI3OutMax=[]  SumI4OutMin=[]  SumI4OutMax=[]  SumDOutMin=[]  SumDOutMax=[]  DifferentiatorOutMin=[]  DifferentiatorOutMax=[]  FilterDiffOutCoefMin=[]  FilterDiffOutCoefMax=[]  ReciprocalOutMin=[]  ReciprocalOutMax=[]  SumDenOutMin=[]  SumDenOutMax=[]  SumNumOutMin=[]  SumNumOutMax=[]  DivideOutMin=[]  DivideOutMax=[]  UdiffTsProdOutMin=[]  UdiffTsProdOutMax=[]  NTsProdOutMin=[]  NTsProdOutMax=[]  UintegralTsProdOutMin=[]  UintegralTsProdOutMax=[]  UngainTsProdOutMin=[]  UngainTsProdOutMax=[]  ClampingZeroOutDataTypeStr=Inherit: Inherit via back propagation  ClampingZeroOutMin=[]  ClampingZeroOutMax=[]  FilterDenConstantOutDataTypeStr=Inherit: Inherit via back propagation  FilterDenConstantOutMin=[]  FilterDenConstantOutMax=[]  PCopyOutDataTypeStr=Inherit: Inherit via back propagation  PCopyOutMin=[]  PCopyOutMax=[]  NCopyOutDataTypeStr=Inherit: Inherit via back propagation  NCopyOutMin=[]  NCopyOutMax=[]  IntegratorContinuousStateAttributes=''  IntegratorStateMustResolveToSignalObject=off  IntegratorRTWStateStorageClass=Auto  FilterContinuousStateAttributes=''  FilterStateMustResolveToSignalObject=off  FilterRTWStateStorageClass=Auto  ParallelPVariant=InternalParameters  IdealPVariant=Disabled  IVariant=InternalParameters  DVariant=InternalParameters  IntegratorVariant=Continuous  SatVariant=Disabled  AWVariant=Passthrough  PCopyVariant=Disabled  TRVariant=Disabled  FdbkBlocksVariant=Forward  IdealPFdbkVariant=Disabled  SatFdbkVariant=Disabled  DerivativeFilterVariant=ContFilter  NVariant=InternalParameters  NCopyVariant=Disabled  FilterICVariant=InternalICsFilter  IntegratorICVariant=InternalICs  ExternalResetVariant=Disabled  TRSumVariant=Passthrough  SumFdbkVariant=Disabled  SumVariant=Sum_PID  TsampFilterVariant=InternalTs  TsampNgainVariant=Passthrough  TsampIntegralVariant=Disabled_SignalSpec  ExternalSaturationOutDataTypeStr=Inherit: Same as second input  DerivativeSourceVariant=ErrorSignal
  Scope : Scope
  Scope1 : Scope
  Sum : Sum  Inputs=|+-
  Sum1 : Sum  Inputs=|+-
  U1d : Outport
  wires:
  PID Controller/1 -> Gain1/1
  Gain/1 -> Sum1/1  "Vzd"
  Sum1/1 -> PID Controller/1  "evz"
  Pz/1 -> Sum/2
  Sum/1 -> Gain/1
  Pzd/1 -> Sum/1
  Gain1/1 -> Add/1
  Vz/1 -> Sum1/2
  Constant/1 -> Scope1/1, Add/2
  Add/1 -> MATLAB Function/1(u)
  MATLAB Function/1(y) -> Scope/1, U1d/1

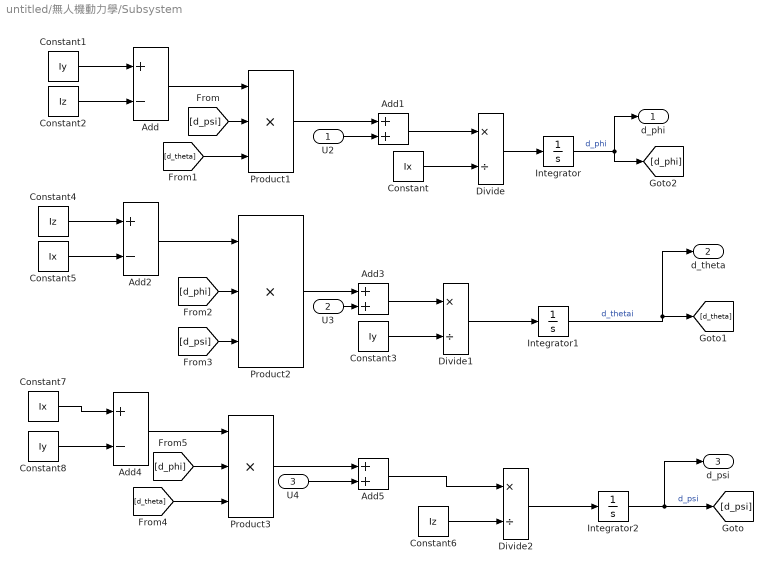
== system untitled/無人機動力學/Subsystem ==
  U2 : Inport
  U3 : Inport  Port=2
  U4 : Inport  Port=3
  Add : Sum  Inputs=+-
  Add1 : Sum
  Add2 : Sum  Inputs=+-
  Add3 : Sum
  Add4 : Sum  Inputs=+-
  Add5 : Sum
  Constant : Constant  Value=Ix
  Constant1 : Constant  Value=Iy
  Constant2 : Constant  Value=Iz
  Constant3 : Constant  Value=Iy
  Constant4 : Constant  Value=Iz
  Constant5 : Constant  Value=Ix
  Constant6 : Constant  Value=Iz
  Constant7 : Constant  Value=Ix
  Constant8 : Constant  Value=Iy
  Divide : Product  Inputs=*/
  Divide1 : Product  Inputs=*/
  Divide2 : Product  Inputs=*/
  Integrator : Integrator
  Integrator1 : Integrator
  Integrator2 : Integrator
  Product1 : Product  Inputs=3
  Product2 : Product  Inputs=3
  Product3 : Product  Inputs=3
  d_phi : Outport
  d_theta : Outport  Port=2
  d_psi : Outport  Port=3
  wires:
  Integrator1/1 -> d_theta/1, [d_theta]  "d_thetai"
  [d_theta] -> Product3/3
  Add/1 -> Product1/1
  Add2/1 -> Product2/1
  [d_phi] -> Product2/2
  Integrator/1 -> [d_phi], d_phi/1  "d_phi"
  U4/1 -> Add5/2
  Product1/1 -> Add1/1
  Add1/1 -> Divide/1
  U3/1 -> Add3/2
  Constant/1 -> Divide/2
  Divide1/1 -> Integrator1/1
  Product3/1 -> Add5/1
  Add5/1 -> Divide2/1
  Constant7/1 -> Add4/1
  Constant5/1 -> Add2/2
  Constant1/1 -> Add/1
  [d_theta] -> Product1/3
  Constant2/1 -> Add/2
  U2/1 -> Add1/2
  [d_psi] -> Product2/3
  Constant4/1 -> Add2/1
  Constant3/1 -> Divide1/2
  Integrator2/1 -> d_psi/1, [d_psi]  "d_psi"
  Product2/1 -> Add3/1
  Add3/1 -> Divide1/1
  Divide2/1 -> Integrator2/1
  Divide/1 -> Integrator/1
  Constant6/1 -> Divide2/2
  Add4/1 -> Product3/1
  Constant8/1 -> Add4/2
  [d_phi] -> Product3/2
  [d_psi] -> Product1/2

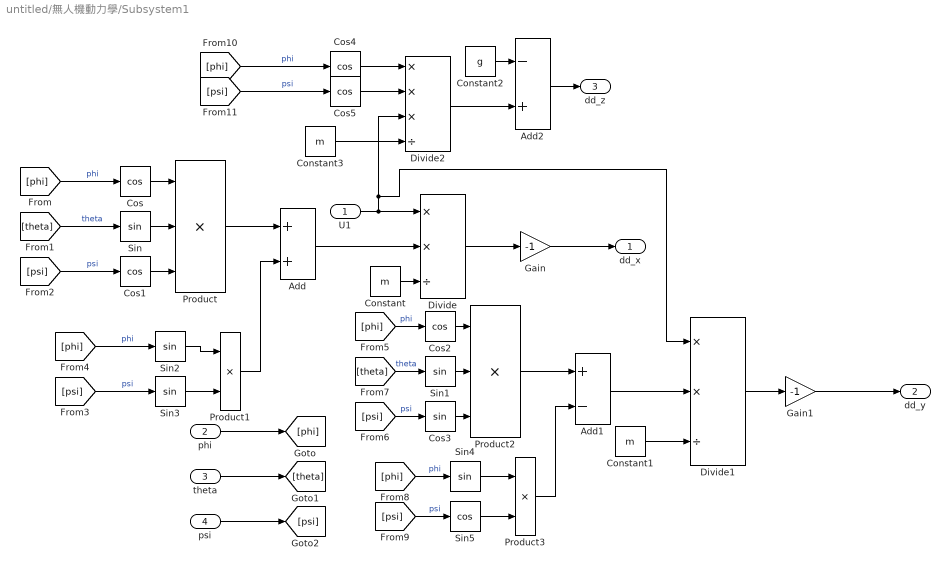
== system untitled/無人機動力學/Subsystem1 ==
  U1 : Inport
  phi : Inport  Port=2
  theta : Inport  Port=3
  psi : Inport  Port=4
  Add : Sum
  Add1 : Sum  Inputs=+-
  Add2 : Sum  Inputs=-+
  Constant : Constant  Value=m  SampleTime=-1
  Constant1 : Constant  Value=m  SampleTime=-1
  Constant2 : Constant  Value=g
  Constant3 : Constant  Value=m  SampleTime=-1
  Cos{,1..2,4..5} (5 alike) : Trigonometry  Operator=cos
  Cos3 : Trigonometry
  Divide : Product  Inputs=**/
  Divide1 : Product  Inputs=**/
  Divide2 : Product  Inputs=***/
  Gain : Gain  Gain=-1
  Gain1 : Gain  Gain=-1
  Product : Product  Inputs=3
  Product1 : Product
  Product2 : Product  Inputs=3
  Product3 : Product
  Sin{,1..4} (5 alike) : Trigonometry
  Sin5 : Trigonometry  Operator=cos
  dd_x : Outport
  dd_y : Outport  Port=2
  dd_z : Outport  Port=3
  wires:
  Divide2/1 -> Add2/2
  [psi] -> Sin3/1  "psi"
  Sin4/1 -> Product3/1
  psi/1 -> [psi]
  [psi] -> Sin5/1  "psi"
  Constant2/1 -> Add2/1
  Gain/1 -> dd_x/1
  Divide/1 -> Gain/1
  Sin2/1 -> Product1/1
  Cos/1 -> Product/1
  [psi] -> Cos5/1  "psi"
  Constant3/1 -> Divide2/4
  Sin1/1 -> Product2/2
  Product2/1 -> Add1/1
  U1/1 -> Divide1/1, Divide2/3, Divide/1
  [theta] -> Sin1/1  "theta"
  [phi] -> Sin4/1  "phi"
  [phi] -> Cos4/1  "phi"
  Cos4/1 -> Divide2/1
  Constant1/1 -> Divide1/3
  [psi] -> Cos3/1  "psi"
  Add/1 -> Divide/2
  Constant/1 -> Divide/3
  [phi] -> Cos2/1  "phi"
  [phi] -> Cos/1  "phi"
  [theta] -> Sin/1  "theta"
  Cos2/1 -> Product2/1
  Product/1 -> Add/1
  Gain1/1 -> dd_y/1
  Product1/1 -> Add/2
  Cos5/1 -> Divide2/2
  Product3/1 -> Add1/2
  Sin3/1 -> Product1/2
  [phi] -> Sin2/1  "phi"
  theta/1 -> [theta]
  Cos1/1 -> Product/3
  Sin/1 -> Product/2
  Add2/1 -> dd_z/1
  Divide1/1 -> Gain1/1
  [psi] -> Cos1/1  "psi"
  Add1/1 -> Divide1/2
  Cos3/1 -> Product2/3
  Sin5/1 -> Product3/2
  phi/1 -> [phi]

== matlab function untitled/高度控制器/MATLAB Function ==
  data: u input; y output
function y = fcn(u)
u(u>20) = 20;
y = u;

== matlab function untitled/混合控制器/MATLAB Function ==
  data: u input; y output
function y = fcn(u)
u(u<0) = 0;
y = u;

== matlab function untitled/位置控制器/MATLAB Function ==
  data: u input; y output
function y = fcn(u)
% 
% y = [cos(u) sin(u);
%     -sin(u) cos(u)];

y = [sin(u) cos(u);
     -cos(u) sin(u)];

== matlab function untitled/位置控制器/MATLAB Function1 ==
  data: u input; y output
function y = fcn(u)
u(u>0.2) = 0.2;
u(u<-0.2) = -0.2;
y = u;

== matlab function untitled/Plant/MATLAB Function ==
  data: T_in input; T_out output; T_max input
function T_out = fcn(T_in, T_max)
% T_in: 4x1 向量，代表矩陣算出來的「期望推力」 (未飽和)
% T_max: 純量，代表單馬達最大推力 (例如 8.829)
% T_out: 4x1 向量，經過「動態調整」後的推力

% 1. 找出四個馬達中，需求最大的那個值
max_thrust_req = max(T_in);

% 2. 計算「超出的量」 (Overshoot)
excess = max_thrust_req - T_max;

% 3. 動態飽和邏輯 (核心)
if excess > 0
    % 如果有馬達超過上限，我們不只是把它「削平」
    % 而是將「所有馬達」都減去這個超出的量。
    % 這樣做可以降低總推力，但「保留馬達之間的差值」。
    % 差值保留了，ROLL/PITCH 的力矩就不會變形！
    T_out = T_in - excess;
else
    % 如果沒超過，就直接通過
    T_out = T_in;
end

% 4. 下限保護 (不能小於 0)
% 經過上述減法後，有些馬達可能會變成負數，這裡做最後的 0 保護
% (這雖然會造成一點點失真，但比上限飽和安全得多)
for i = 1:4
    if T_out(i) < 0
        T_out(i) = 0;
    end
end

% 5. 再次上限保護 (以防萬一)
% 經過上述處理，理論上不會超過 T_max，但加一層保險
for i = 1:4
    if T_out(i) > T_max
        T_out(i) = T_max;
    end
end

== matlab function untitled/姿態控制器/MATLAB Function ==
  settings: updateMethod=DISCRETE
  data: cmd input; u_control output; y_actual input; dt input; Kp_new output; Ki_new output; Kd_new output
function [u_control, Kp_new, Ki_new, Kd_new] = fcn_MRAC_Lyapunov(cmd, y_actual, dt)
    % cmd:      期望輸入 (例如 wd, 圖中的期望角速度)
    % y_actual: 實際輸出 (例如 d_phi, 圖中的實際角速度)
    % dt:       採樣時間 (例如 0.001 或 0.01，需與模擬步長一致)
    
    % === 1. 參數設定 (Tunable Parameters) ===
    % -----------------------------------
    % A. 參考模型參數 (理想的二階系統 response)
    wn = 10;        % 自然頻率 (越大反應越快)
    zeta = 0.707;   % 阻尼比 (0.707 為標準不震盪)
    
    % B. 自適應增益 (Adaptation Rate - Gamma)
    % 決定參數調整的快慢，太快會震盪，太慢沒效果
    gam_p = 0;    
    gam_i = 0;
    gam_d = 0; 
    
    % C. PID 參數的初始值與限制 (防止參數發散)
    Kp_init = 1.0;  Kp_max = 20; Kp_min = 0.1;
    Ki_init = 0.01;  Ki_max = 10; Ki_min = 0.0;
    Kd_init = 0.5;  Kd_max = 5;  Kd_min = 0.0;
    
    % === 2. 變數初始化 (Persistent Memory) ===
    % -----------------------------------
    % 這些變數會記住上一次呼叫的值
    persistent xm_1 xm_2        % 參考模型狀態 (位置, 速度)
    persistent e_integral       % PID 的誤差積分項
    persistent prev_error       % 用於計算微分項
    persistent Kp Ki Kd         % 當前的 PID 參數
    
    if isempty(xm_1)
        xm_1 = 0; xm_2 = 0;
        e_integral = 0;
        prev_error = 0;
        Kp = Kp_init; Ki = Ki_init; Kd = Kd_init;
    end
    
    % === 3. 執行參考模型 (Reference Model Dynamics) ===
    % -----------------------------------
    % 使用尤拉法 (Euler Integration) 模擬理想系統
    % 理想方程式: y_m'' + 2*zeta*wn*y_m' + wn^2*y_m = wn^2*r
    
    u_model = wn^2 * cmd;
    dxm_2 = -2*zeta*wn*xm_2 - wn^2*xm_1 + u_model; % 加速度
    
    xm_2 = xm_2 + dxm_2 * dt;   % 更新理想速度
    xm_1 = xm_1 + xm_2 * dt;    % 更新理想位置 (輸出 ym)
    
    y_model = xm_1;             % 這是我們希望無人機做到的輸出
    
    % === 4. 計算誤差訊號 (Error Signals) ===
    % -----------------------------------
    % 追蹤誤差 (Tracking Error): 實際與理想的差距 -> 用來調整參數
    e_track = y_actual - y_model; 
    
    % 控制誤差 (Control Error): 期望與實際的差距 -> 用來計算 PID 輸出
    e_control = cmd - y_actual;
    
    % 計算 PID 需要的三個訊號向量 (Regressor Vector phi)
    % P項訊號
    phi_p = e_control;
    
    % I項訊號 (對控制誤差積分)
    e_integral = e_integral + e_control * dt;
    phi_i = e_integral;
    
    % D項訊號 (對控制誤差微分)
    phi_d = (e_control - prev_error) / dt;
    prev_error = e_control;
    
    % === 5. Lyapunov 參數更新律 (Adaptation Law) ===
    % -----------------------------------
    % 基本公式: dK/dt = -Gamma * e_track * phi * P_lyap
    % 這裡簡化 P_lyap 為正值，負號代表負回授修正
    
    % 注意：這裡的正負號取決於系統方向，若誤差變大，我們需要參數變大還是變小？
    % 對於標準正增益系統，通常使用以下形式：
    
    dKp = -gam_p * e_track * phi_p; 
    dKi = -gam_i * e_track * phi_i;
    dKd = -gam_d * e_track * phi_d;
    
    % 更新參數 (積分)
    Kp = Kp + dKp * dt;
    Ki = Ki + dKi * dt;
    Kd = Kd + dKd * dt;
    
    % 強制限制參數範圍 (Projection / Saturation) - 關鍵步驟！
    Kp = max(min(Kp, Kp_max), Kp_min);
    Ki = max(min(Ki, Ki_max), Ki_min);
    Kd = max(min(Kd, Kd_max), Kd_min);
    
    % === 6. 計算最終控制輸出 (Control Law) ===
    % -----------------------------------
    u_control = Kp*phi_p + Ki*phi_i + Kd*phi_d;
    
    % 輸出新的參數供觀察
    Kp_new = Kp;
    Ki_new = Ki;
    Kd_new = Kd;

end

== matlab function untitled/Plant/MATLAB Function2 ==
  data: T1 input; X output
function X = thrust_to_pwm(T1)
%#codegen
% 由推力 T1 (N) 計算對應 PWM 百分比 X (%)
% 方程式: T1*1000 = 964.308*X - 211.41

X = (T1 * 200 + 211.41) / 964.308;
X = max(0, min(X, 100));   % 限制在 0~100% 之間

end
